simulink model "GasBench"  (R2026b)
settings: Solver=ode23t  StopTime=0.2  RelTol=1e-5
values from neighbouring files (symbols this model uses):
  P = struct('finger', fi, 'gas', ga, 'obj', o, 'bench', b)    [gripperBenchParams.m]
libraries: fl_lib x9, nesl_utility x1
settings Model: Creator=amavromm  LastModifiedBy=amavromm
settings SimscapeCC: SimscapeLogType=all  SimscapeNominalValues="[{\"value\":\"1\",\"unit\":\"A\"},{\"value\":\"1\",\"unit\":\"bar\"},{\"value\":\"1\",\"unit\":\"cm^2\"},{\"value\":\"1\",\"unit\":\"cm^3/s\"},{\"value\":\"1\",\"unit\":\"kJ/kg\"},{\"value\":\"1\",\"unit\":\"kW\"},{\"value\":\"1\",\"unit\":\"l\"},{\"value\":\"1\",\"unit\":\"N\"},{\"value\":\"1\",\"unit\":\"N*m\"},{\"value\":\"1\",\"unit\":\"V\"},{\"value\":\"0.001\",\"unit\":\"Wb\"}]"  SimscapeUseEnergyAccounting=off

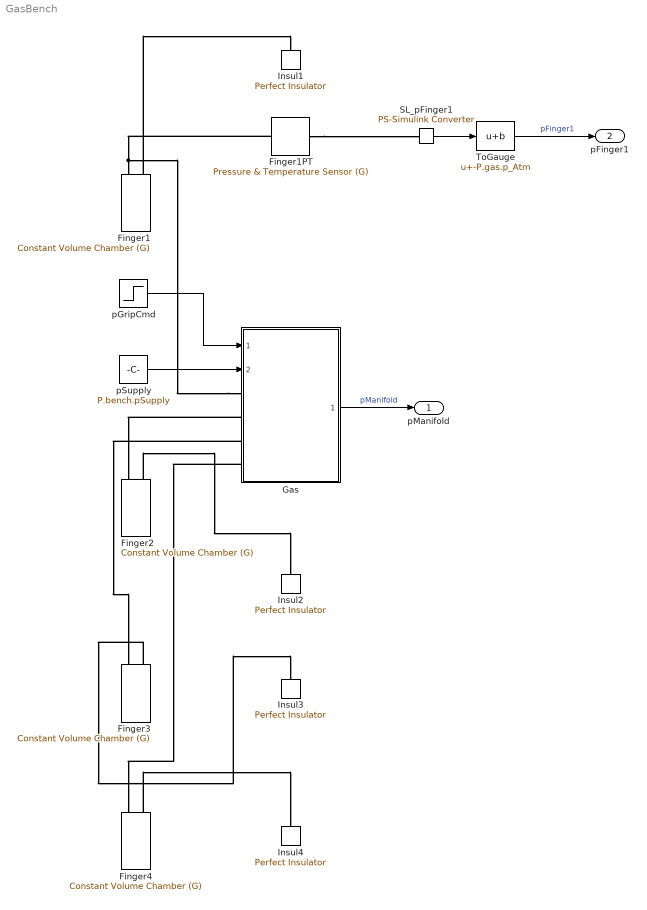
== system GasBench ==
  Finger{1..4} (4 alike) : fl_lib/Gas/Elements/Constant Volume Chamber (G)  volume=P.gas.V_Finger0 m^3  num_ports=1  area_A=pi/4*P.gas.d_Tube^2 m^2  area_B=0.01 m^2  area_C=0.01 m^2  area_D=0.01 m^2  p_I_specify=on  p_I_priority=High  p_I=P.gas.p_Atm + P.gas.p_Init Pa  p_I_nominal_specify=off  p_I_nominal_value=1  p_I_nominal_unit=MPa  T_I_specify=on  T_I_priority=High  T_I=P.gas.T_Amb K  T_I_nominal_specify=off  T_I_nominal_value=1  T_I_nominal_unit=K  rho_I_specify=off  rho_I_priority=None  rho_I=1.2 kg/m^3  rho_I_nominal_specify=off  rho_I_nominal_value=1  rho_I_nominal_unit=kg/m^3
  Finger1PT : fl_lib/Gas/Sensors/Pressure & Temperature Sensor (G)  reference=foundation.enum.MeasurementReference.absolute  pressure=true  pressure_spec=foundation.enum.PressureMeasementSpec.Absolute  temperature=false
  Gas : Subsystem  ReferencedSubsystem=GripperGas
  Insul{1..4} (4 alike) : fl_lib/Thermal/Thermal Elements/Perfect Insulator  T_specify=off  T_priority=None  T=293.15 K  T_nominal_specify=off  T_nominal_value=1  T_nominal_unit=K
  SL_pFinger1 : nesl_utility/PS-Simulink Converter  PhysicalDomain=network_engine_domain  SubClassName=ps_output  LeftPortType=input  RightPortType=output  PseudoPeriodic=off  Frequencies=[]  VectorFormat=inherit  Unit=Pa  AffineConversion=off
  ToGauge : Bias  Bias=-P.gas.p_Atm  SaturateOnIntegerOverflow=off
  pGripCmd : Step  Time=P.bench.tStep  FinalValue=P.bench.pCmd  SampleTime=0
  pSupply : Constant  Value=P.bench.pSupply
  pManifold : Outport
  pFinger1 : Outport  Port=2
  wires:
  pGripCmd/1 -> Gas/1
  pSupply/1 -> Gas/2
  Gas/1 -> pManifold/1  "pManifold"
  SL_pFinger1/1 -> ToGauge/1
  ToGauge/1 -> pFinger1/1  "pFinger1"
  connections:
  Gas/LConn1 -- Finger1PT/LConn1 -- Finger1/LConn1
  Gas/LConn2 -- Finger2/LConn1
  Gas/LConn3 -- Finger3/LConn1
  Gas/LConn4 -- Finger4/LConn1
  Finger1/LConn2 -- Insul1/LConn1
  Finger2/LConn2 -- Insul2/LConn1
  Finger3/LConn2 -- Insul3/LConn1
  Finger4/LConn2 -- Insul4/LConn1
  Finger1PT/RConn1 -- SL_pFinger1/LConn1
